simulink model "sm_car_"  (R2026b)
settings: Solver=ode23t  StopTime=100  MaxStep=0.4  AbsTol=1e-3  EnableMultiTasking=on
PreLoadFcn:
  | % Due to usability issue in Repeating Sequence block
  | warning('off','Simulink:Masking:Invalid');
  | 
  | % Eliminate unnecessary warnings in inactive variants
  | % Warnings generated only if you click through inactive variant
  | warning('off','MATLAB:nonExistentField');
  | warning('off','Simulink:Parameters:BlkParamUndefined');
PostLoadFcn:
  | set_param([bdroot '/Vehicle'],'popup_trailer','Off')
  | warning('off','sm:sli:setup:compile:LocalSolverNotSupported')
  | %sm_car_config_maneuver(bdroot,'WOT Braking');
  | sm_car_config_vehicle(bdroot,'false');
  | sm_car_config_logging(bdroot);
InitFcn:
  | sm_car_config_camera;
  | Vehicle = sm_car_vehcfg_checkConfig(Vehicle);
  | sm_car_check_tire_model(bdroot);
StartFcn:
  | tic;
StopFcn:
  | Elapsed_Sim_Time = toc;
  | % disp(['Elapsed Sim Time = ' num2str(Elapsed_Sim_Time)]);
undefined symbols (not defined in the file or in its folder): acc_theta, accel_ramp_rate, Axle1D, AxleIn, Camera, Control, Driver, Init, Maneuver, Pedal, Scene, ShaftL1, ShaftL2, ShaftR1, ShaftR2, Visual, X, xy_data_car_side, Y, Z
libraries: sm_lib x290, fl_lib x171, nesl_utility x144, simulink x60, simulink_extras x14, sdl_lib x14, SimscapeFluids_lib x7, Damper_Element x4, Tire_1x2x x4, ee_lib x3, Scene_Utilities x3, sharedTrackingLibrary x2
(part 6 of 22)

== system sm_car_/Controller/TrqVec_FLC/Power Control ==
  rAccelPedal : Inport
  VehBus : Inport  Port=2
  aSteerWheel : Inport  Port=3
  Bus Creator : BusCreator  Inputs=2
  Bus Selector : BusSelector  OutputSignals=Chassis.Body.CG.vx,Chassis.Body.CG.gy,Chassis.Body.CG.nYaw,Power.MotorL2.w,Power.MotorR2.w
  Gain : Gain  Gain=max(Control.MotorTrq)
  Gain1 : Gain  Gain=max(Control.MotorTrq)
  Gain2 : Gain  Gain=1/9.80665
  TV_FLC : Subsystem  TreatAsAtomicUnit=on  ReferencedSubsystem=TV_FLC  StrWheelRatio=Control.StrWheelRatio  Ku=Control.UndersteerGradient  L=Control.Wheelbase  rwheel=Control.WheelRad  Gr=Control.GearRatio  fis=Control.FuzzySystem  Kp=250  tr=Control.RearTrack  alpha_max=Control.SlipTh  MotorT=Control.MotorTrq  MotorW=Control.MotorW  F=Control.F  Tmax=max(Control.MotorTrq)
  Power : Outport  VectorParamsAs1DForOutWhenUnconnected=off
  wires:
  VehBus/1 -> Bus Selector/1
  Bus Selector/1 -> TV_FLC/2  "<vx>"
  Bus Selector/2 -> Gain2/1  "<gy>"
  Bus Selector/3 -> TV_FLC/4  "<nYaw>"
  Bus Selector/4 -> TV_FLC/5  "<w>"
  Bus Selector/5 -> TV_FLC/6  "<w>"
  rAccelPedal/1 -> TV_FLC/7  "Throttle[~]"
  Bus Creator/1 -> Power/1
  TV_FLC/1 -> Gain/1  "MMotorL2Demand"
  TV_FLC/2 -> Gain1/1  "MMotorR2Demand"
  Gain/1 -> Bus Creator/1  "MMotorL2Demand"
  Gain1/1 -> Bus Creator/2  "MMotorR2Demand"
  Gain2/1 -> TV_FLC/3
  aSteerWheel/1 -> TV_FLC/1

== system sm_car_/Controller/TrqVec_FLC/Spring Damper ==
  Bus Creator : BusCreator  Inputs=4
  Bus Creator1 : BusCreator  Inputs=4
  Constant : Constant  Value=[0 0 0 0]
  Constant1 : Constant  Value=[0 0 0 0]
  Demux : Demux
  Demux1 : Demux
  Damper : Outport  VectorParamsAs1DForOutWhenUnconnected=off
  Spring : Outport  Port=2  VectorParamsAs1DForOutWhenUnconnected=off
  wires:
  Constant/1 -> Demux/1
  Demux/3 -> Bus Creator/3  "L2"
  Demux/4 -> Bus Creator/4  "R2"
  Demux/1 -> Bus Creator/1  "L1"
  Demux/2 -> Bus Creator/2  "R1"
  Demux1/2 -> Bus Creator1/2  "R1"
  Demux1/1 -> Bus Creator1/1  "L1"
  Demux1/4 -> Bus Creator1/4  "R2"
  Demux1/3 -> Bus Creator1/3  "L2"
  Constant1/1 -> Demux1/1
  Bus Creator1/1 -> Damper/1  "Damper"
  Bus Creator/1 -> Spring/1  "Spring"

== system sm_car_/Controller/TrqVec_FLC/Susp ==
  aSteerWheel : Inport
  vx : Inport  Port=2
  1-D Lookup Table : Lookup_n-D  NumberOfTableDimensions=1  BreakpointsForDimension1=Steer.Gain.vVehicle.Value  Table=Steer.Gain.n.Value  InterpMethod=Linear Lagrange  InternalRulePriority=Speed  RndMeth=Simplest
  Bus Creator{1..4} (4 alike) : BusCreator  Inputs=1
  Gain : Gain  Gain=3.6
  Product : Product
  Saturation : Saturate  UpperLimit=Steer.Limits.aUpper.Value  LowerLimit=Steer.Limits.aLower.Value  LinearizeAsGain=off  ZeroCross=off
  Transfer Fcn (with initial states) : simulink_extras/Additional Linear/Transfer Fcn (with initial states)  N=[1]  D="[1/Steer.fActuatorCutoff.Value  1]"  X0=-1
  SuspA1 : Outport  VectorParamsAs1DForOutWhenUnconnected=off
  SuspA2 : Outport  Port=2  VectorParamsAs1DForOutWhenUnconnected=off
  wires:
  Bus Creator4/1 -> Bus Creator1/1  "Steer"
  Bus Creator2/1 -> Bus Creator3/1  "Steer"
  Bus Creator3/1 -> SuspA2/1  "SuspA2"
  Bus Creator1/1 -> SuspA1/1  "SuspA1"
  aSteerWheel/1 -> Product/1, Bus Creator4/1  "aSteerWheel"
  Saturation/1 -> Bus Creator2/1  "aSteerWheel"
  vx/1 -> Gain/1
  Transfer Fcn (with initial states)/1 -> Product/2
  Product/1 -> Saturation/1
  Gain/1 -> 1-D Lookup Table/1
  1-D Lookup Table/1 -> Transfer Fcn (with initial states)/1

== system sm_car_/Controller/TrqVec_FLC_V2/Brake Control ==
  "rBrakePedal " : Inport
  "VehBus " : Inport  Port=2
  Pedal : Subsystem  VariantControl=Pedal
  " Brakes" : Outport  VectorParamsAs1DForOutWhenUnconnected=off

== system sm_car_/Controller/TrqVec_FLC_V2/Driveline Control ==
  Bus Creator : BusCreator  Inputs=1
  Constant : Constant  Value=0
  Driveline : Outport  VectorParamsAs1DForOutWhenUnconnected=off
  wires:
  Constant/1 -> Bus Creator/1  "placeholder"
  Bus Creator/1 -> Driveline/1  "Driveline"

== system sm_car_/Controller/TrqVec_FLC_V2/Power Control ==
  rAccelPedal : Inport
  VehBus : Inport  Port=2
  aSteerWheel : Inport  Port=3
  Bus Creator : BusCreator  Inputs=2
  Bus Selector : BusSelector  OutputSignals=Chassis.Body.CG.vx,Chassis.Body.CG.gx,Chassis.Body.CG.gy,Chassis.Body.CG.nYaw,Chassis.SuspA2.LinkageL.Upright.Upright.w,Chassis.SuspA2.LinkageR.Upright.Upright.w,Chassis.Body.CG.vy
  Controler type : Constant  Value=2
  Gain : Gain  Gain=max(Control.MotorTrq)
  Gain1 : Gain  Gain=max(Control.MotorTrq)
  Gain2 : Gain  Gain=1/9.80665
  TV FLC V2 : Subsystem  TreatAsAtomicUnit=on  ReferencedSubsystem=TV_FLC_V2  MotorT=Control.MotorTrq  Gr=Control.GearRatio  MotorW=Control.MotorW  rwheel=Control.WheelRad  tr=Control.RearTrack  a=Control.FrontTrackToCG  a_cop=Control.FrontTrackToCoP  Af=Control.FrontalArea  cd=Control.LiftCoef  g=Control.GravitationalAcc  ro=Control.AirDensity  m=Control.Mass  h_CG=Control.CGHeight  L=Control.Wheelbase  Gain=Control.StrWheelRatio  Ku=Control.UndersteerGradient  F=Control.F  P=Control.Proportional_P  I=Control.Integral_I  D=Control.Derivative_D  N=Control.Filter_N  Load_Ref=Control.LoadRef  Slip_Ref=Control.SlipRef  FIS_1=Control.FuzzySystem_1  FIS_2=Control.FuzzySystem_2  FIS_3=Control.FuzzySystem_3  vx_th=Control.ActivationVelocity  Tmax=max(Control.MotorTrq)  C_alpha_F=Control.CalphaF
  Power : Outport  VectorParamsAs1DForOutWhenUnconnected=off
  wires:
  aSteerWheel/1 -> TV FLC V2/1
  Gain2/1 -> TV FLC V2/4
  Gain1/1 -> Bus Creator/2  "MMotorR2Demand"
  Gain/1 -> Bus Creator/1  "MMotorL2Demand"
  TV FLC V2/2 -> Gain1/1  "MMotorR2Demand"
  TV FLC V2/1 -> Gain/1  "MMotorL2Demand"
  Bus Creator/1 -> Power/1
  rAccelPedal/1 -> TV FLC V2/9  "Throttle[~]"
  Bus Selector/6 -> TV FLC V2/7  "<w>"
  Bus Selector/5 -> TV FLC V2/6  "<w>"
  Bus Selector/4 -> TV FLC V2/5  "<nYaw>"
  Bus Selector/3 -> Gain2/1  "<gy>"
  Bus Selector/1 -> TV FLC V2/2  "<vx>"
  VehBus/1 -> Bus Selector/1
  Bus Selector/2 -> TV FLC V2/3  "<gx>"
  Bus Selector/7 -> TV FLC V2/8  "<vy>"
  Controler type/1 -> TV FLC V2/10

== system sm_car_/Controller/TrqVec_FLC_V2/Spring Damper ==
  Bus Creator : BusCreator  Inputs=4
  Bus Creator1 : BusCreator  Inputs=4
  Constant : Constant  Value=[0 0 0 0]
  Constant1 : Constant  Value=[0 0 0 0]
  Demux : Demux
  Demux1 : Demux
  Damper : Outport  VectorParamsAs1DForOutWhenUnconnected=off
  Spring : Outport  Port=2  VectorParamsAs1DForOutWhenUnconnected=off
  wires:
  Bus Creator/1 -> Spring/1  "Spring"
  Bus Creator1/1 -> Damper/1  "Damper"
  Constant1/1 -> Demux1/1
  Demux1/3 -> Bus Creator1/3  "L2"
  Demux1/4 -> Bus Creator1/4  "R2"
  Demux1/1 -> Bus Creator1/1  "L1"
  Demux1/2 -> Bus Creator1/2  "R1"
  Demux/2 -> Bus Creator/2  "R1"
  Demux/1 -> Bus Creator/1  "L1"
  Demux/4 -> Bus Creator/4  "R2"
  Demux/3 -> Bus Creator/3  "L2"
  Constant/1 -> Demux/1

== system sm_car_/Controller/TrqVec_FLC_V2/Susp ==
  aSteerWheel : Inport
  vx : Inport  Port=2
  1-D Lookup Table : Lookup_n-D  NumberOfTableDimensions=1  BreakpointsForDimension1=Steer.Gain.vVehicle.Value  Table=Steer.Gain.n.Value  InterpMethod=Linear Lagrange  InternalRulePriority=Speed  RndMeth=Simplest
  Bus Creator{1..4} (4 alike) : BusCreator  Inputs=1
  Gain : Gain  Gain=3.6
  Product : Product
  Saturation : Saturate  UpperLimit=Steer.Limits.aUpper.Value  LowerLimit=Steer.Limits.aLower.Value  LinearizeAsGain=off  ZeroCross=off
  Transfer Fcn (with initial states) : simulink_extras/Additional Linear/Transfer Fcn (with initial states)  N=[1]  D="[1/Steer.fActuatorCutoff.Value  1]"  X0=-1
  SuspA1 : Outport  VectorParamsAs1DForOutWhenUnconnected=off
  SuspA2 : Outport  Port=2  VectorParamsAs1DForOutWhenUnconnected=off
  wires:
  1-D Lookup Table/1 -> Transfer Fcn (with initial states)/1
  Gain/1 -> 1-D Lookup Table/1
  Product/1 -> Saturation/1
  Transfer Fcn (with initial states)/1 -> Product/2
  vx/1 -> Gain/1
  Saturation/1 -> Bus Creator2/1  "aSteerWheel"
  aSteerWheel/1 -> Bus Creator4/1, Product/1  "aSteerWheel"
  Bus Creator1/1 -> SuspA1/1  "SuspA1"
  Bus Creator3/1 -> SuspA2/1  "SuspA2"
  Bus Creator2/1 -> Bus Creator3/1  "Steer"
  Bus Creator4/1 -> Bus Creator1/1  "Steer"

== system sm_car_/Controller/TrqVec_FLC_V3/Brake Control ==
  "rBrakePedal " : Inport
  "VehBus " : Inport  Port=2
  Pedal : Subsystem  VariantControl=Pedal
  " Brakes" : Outport  VectorParamsAs1DForOutWhenUnconnected=off

== system sm_car_/Controller/TrqVec_FLC_V3/Driveline Control ==
  Bus Creator : BusCreator  Inputs=1
  Constant : Constant  Value=0
  Driveline : Outport  VectorParamsAs1DForOutWhenUnconnected=off
  wires:
  Bus Creator/1 -> Driveline/1  "Driveline"
  Constant/1 -> Bus Creator/1  "placeholder"

== system sm_car_/Controller/TrqVec_FLC_V3/Power Control ==
  rAccelPedal : Inport
  VehBus : Inport  Port=2
  aSteerWheel : Inport  Port=3
  Bus Creator : BusCreator  Inputs=2
  Bus Selector : BusSelector  OutputSignals=Chassis.SuspA2.LinkageL.Upright.Upright.w,Chassis.SuspA2.LinkageR.Upright.Upright.w
  Bus Selector1 : BusSelector  OutputSignals=v_x,a_x,a_y,phi_dot,v_y
  Data Type Conversion{,1..8} (9 alike) : DataTypeConversion  OutDataTypeStr=single  SaturateOnIntegerOverflow=off  RndMeth=Floor
  Data Type Conversion10 : DataTypeConversion  OutDataTypeStr=double  SaturateOnIntegerOverflow=off  RndMeth=Floor
  Data Type Conversion11 : DataTypeConversion  OutDataTypeStr=double  SaturateOnIntegerOverflow=off  RndMeth=Floor
  Gain : Gain  Gain=max(Control.MotorTrq)
  Gain1 : Gain  Gain=max(Control.MotorTrq)
  State Estimation : Subsystem
  TV FLC V3 : Subsystem  TreatAsAtomicUnit=on  ReferencedSubsystem=TV_FLC_V3  MotorT=Control.MotorTrq  Gr=Control.GearRatio  MotorW=Control.MotorW  rwheel=Control.WheelRad  tr=Control.RearTrack  a=Control.FrontTrackToCG  a_cop=Control.FrontTrackToCoP  Af=Control.FrontalArea  cd=Control.LiftCoef  Value=Control.GravitationalAcc  ro=Control.AirDensity  m=Control.Mass  h_CG=Control.CGHeight  L=Control.Wheelbase  StrWhlR=Control.StrWheelRatio  Ku=Control.UndersteerGradient  F=Control.F  Slip_Ctrl_Kp=70  Slip_Ctrl_Ki=150  Slip_Ctrl_Kd=1.5  Slip_Ctrl_Kn=Control.Filter_N  Load_Ref=Control.LoadRef  Slip_Ref=Control.SlipRef  FIS=Control.FuzzySystem  vx_th=Control.ActivationVelocity  Tmax=max(Control.MotorTrq)  C_alpha_F=Control.CalphaF  Slip_Steer_th=10  Kp_TV_Yaw=Control.Kp_Yaw  Kp_TV_Beta=Control.Kp_beta
  Power : Outport  VectorParamsAs1DForOutWhenUnconnected=off
  Out Bus Element : Outport  Port=2  PortName=Meas  Element=DYC
  Out Bus Element1 : Outport  Port=2  PortName=Meas  Element=UKF
  wires:
  VehBus/1 -> State Estimation/2(VehBus), Bus Selector/1
  Bus Selector/1 -> Data Type Conversion5/1  "<w>"
  Bus Selector/2 -> Data Type Conversion6/1  "<w>"
  rAccelPedal/1 -> Data Type Conversion8/1  "Throttle[~]"
  Bus Creator/1 -> Power/1
  TV FLC V3/1 -> Data Type Conversion10/1
  Gain/1 -> Bus Creator/1  "MMotorL2Demand"
  Gain1/1 -> Bus Creator/2  "MMotorR2Demand"
  aSteerWheel/1 -> State Estimation/1(aSteerWheel), Data Type Conversion/1
  TV FLC V3/2 -> Data Type Conversion11/1
  Data Type Conversion/1 -> TV FLC V3/1
  Data Type Conversion1/1 -> TV FLC V3/2
  Data Type Conversion2/1 -> TV FLC V3/3
  Data Type Conversion3/1 -> TV FLC V3/4
  Data Type Conversion4/1 -> TV FLC V3/5
  Data Type Conversion5/1 -> TV FLC V3/7
  Data Type Conversion6/1 -> TV FLC V3/8
  Data Type Conversion7/1 -> TV FLC V3/6
  Data Type Conversion8/1 -> TV FLC V3/9
  Data Type Conversion10/1 -> Gain/1
  Data Type Conversion11/1 -> Gain1/1
  TV FLC V3/3 -> Out Bus Element/1
  State Estimation/1(StateEst) -> Bus Selector1/1
  Bus Selector1/1 -> Data Type Conversion1/1  "<v_x>"
  Bus Selector1/4 -> Data Type Conversion4/1  "<phi_dot>"
  Bus Selector1/2 -> Data Type Conversion2/1  "<a_x>"
  Bus Selector1/3 -> Data Type Conversion3/1  "<a_y>"
  Bus Selector1/5 -> Data Type Conversion7/1  "<v_y>"
  State Estimation/2(Meas) -> Out Bus Element1/1  "Estimation"

== system sm_car_/Controller/TrqVec_FLC_V3/Spring Damper ==
  Bus Creator : BusCreator  Inputs=4
  Bus Creator1 : BusCreator  Inputs=4
  Constant : Constant  Value=[0 0 0 0]
  Constant1 : Constant  Value=[0 0 0 0]
  Demux : Demux
  Demux1 : Demux
  Damper : Outport  VectorParamsAs1DForOutWhenUnconnected=off
  Spring : Outport  Port=2  VectorParamsAs1DForOutWhenUnconnected=off
  wires:
  Constant/1 -> Demux/1
  Demux/3 -> Bus Creator/3  "L2"
  Demux/4 -> Bus Creator/4  "R2"
  Demux/1 -> Bus Creator/1  "L1"
  Demux/2 -> Bus Creator/2  "R1"
  Demux1/2 -> Bus Creator1/2  "R1"
  Demux1/1 -> Bus Creator1/1  "L1"
  Demux1/4 -> Bus Creator1/4  "R2"
  Demux1/3 -> Bus Creator1/3  "L2"
  Constant1/1 -> Demux1/1
  Bus Creator1/1 -> Damper/1  "Damper"
  Bus Creator/1 -> Spring/1  "Spring"

== system sm_car_/Controller/TrqVec_FLC_V3/Susp ==
  aSteerWheel : Inport
  vx : Inport  Port=2
  1-D Lookup Table : Lookup_n-D  NumberOfTableDimensions=1  BreakpointsForDimension1=Steer.Gain.vVehicle.Value  Table=Steer.Gain.n.Value  InterpMethod=Linear Lagrange  InternalRulePriority=Speed  RndMeth=Simplest
  Bus Creator{1..4} (4 alike) : BusCreator  Inputs=1
  Gain : Gain  Gain=3.6
  Product : Product
  Saturation : Saturate  UpperLimit=Steer.Limits.aUpper.Value  LowerLimit=Steer.Limits.aLower.Value  LinearizeAsGain=off  ZeroCross=off
  Transfer Fcn (with initial states) : simulink_extras/Additional Linear/Transfer Fcn (with initial states)  N=[1]  D="[1/Steer.fActuatorCutoff.Value  1]"  X0=-1
  SuspA1 : Outport  VectorParamsAs1DForOutWhenUnconnected=off
  SuspA2 : Outport  Port=2  VectorParamsAs1DForOutWhenUnconnected=off
  wires:
  Bus Creator4/1 -> Bus Creator1/1  "Steer"
  Bus Creator2/1 -> Bus Creator3/1  "Steer"
  Bus Creator3/1 -> SuspA2/1  "SuspA2"
  Bus Creator1/1 -> SuspA1/1  "SuspA1"
  aSteerWheel/1 -> Product/1, Bus Creator4/1  "aSteerWheel"
  Saturation/1 -> Bus Creator2/1  "aSteerWheel"
  vx/1 -> Gain/1
  Transfer Fcn (with initial states)/1 -> Product/2
  Product/1 -> Saturation/1
  Gain/1 -> 1-D Lookup Table/1
  1-D Lookup Table/1 -> Transfer Fcn (with initial states)/1

== system sm_car_/Driver/Closed Loop/Driver ==
  vx : Inport
  Ref : Inport  Port=2
  CurPose : Inport  Port=3
  Abs : Abs  SaturateOnIntegerOverflow=off
  Bus Creator5 : BusCreator  Inputs=4
  Bus Selector1 : BusSelector  OutputSignals=vTarget
  Constant : Constant
  Constant1 : Constant  Value=0.8
  Constant9 : Constant  Value=0
  Filter Steer Cmd : TransferFcn  Numerator=[5.7]  Denominator=[1/Driver.Lateral.fSteerCutoff.Value 1]
  Gain4 : Gain  Gain=pi/180
  Get Pose : Subsystem
  Lateral Controller Stanley : drivingvehiclecontroller/Lateral Controller Stanley  ModelType=Kinematic bicycle model  PositionGainF=0.7  PositionGainR=Driver.Lateral.Stanley.NForward.Value  YawRateGain=0.2  DelayGain=0.2  VehicleMass=1575  Lf=1.2  Lr=1.6  TireStiffness=19000  Wheelbase=1.578  MaxSteeringAngle=27
  Longitudinal Driver : autolibshared/Longitudinal Driver  extAccelOvr=off  extDecelOvr=off  extAccelHld=off  extDecelHld=off  extAccelZero=off  extDecelZero=off  cntrlType=Predictive  shftType=None  velUnits=m/s  gearOut=off  Kp=15  Ki=1  Kff=.05  Kg=.01  VehVelVec=[0 100]  KffVec=[.1 .1]  KpVec=[10 10]  KiVec=[5 5]  KgVec=[0 0]  m=320  Kpt=Driver.Long.FTractive.Value  tau=Driver.Long.tDriver.Value  L=3  aR=Driver.Long.NDragRoll.Value  bR=Driver.Long.NDragAero.Value  cR=Driver.Long.NDragAero.Value  g=Driver.Long.gGravity.Value  vnom=100  Kaw=.1  tauerr=.03  tauPt=2  GearInit=0  tShift=.1  pdlVec=[0.1 0.4 0.5 0.9]  upShftTbl=[-1 12.9375 26.4375 39.9375 51.18749999999999 62.4375 72.84375 83.25;-1 16.3125 29.8125 43.3125 54.5624 65.8125 76.78125 87.75;-1 19.6875 33.1875 46.68749999999999 57.9375 69.1875 80.71875 92.25;-1 33 52.5 77.25 100.5 138.75 161.875 185]  dwnShftTbl=[1 9.5625 23.0625 36.5625 47.8125 59.0625 68.90625 78.75;1 12.9375 26.4375 39.9375 51.18749999999999 62.4375 72.84375 83.25;1 16.3125 29.8125 43.3125 54.562499 65.8125 76.78125 87.75;1 19.6875 33.1875 46.68749999999999 57.9375 69.1875 80.71875 92.25]  tClutch=.5  tRev=.5  tPark=120  aMode=1  UpGearVec="[0  1  2  3  4  5  6  7]"  DownGearVec="[1  2  3  4  5  6  7  8]"
  Saturation : Saturate  UpperLimit=inf  LowerLimit=1e-9  ZeroCross=off
  Saturation1 : Saturate  UpperLimit=1  LowerLimit=0  ZeroCross=off
  Saturation2 : Saturate  UpperLimit=1  LowerLimit=0  ZeroCross=off
  Scope : Scope
      settings: ActiveDisplayYMinimum=-1  ActiveDisplayYMaximum=1  DataLoggingVariableName=ScopeData8
  Terminator : Terminator
  Terminator4 : Terminator
  Transfer Fcn : TransferFcn  Denominator=[1/(Driver.Long.fAccelCutoff.Value) 1]
  Transfer Fcn1 : TransferFcn  Denominator=[1/(Driver.Long.fBrakeCutoff.Value) 1]
  DrvBus : Outport  VectorParamsAs1DForOutWhenUnconnected=off
  wires:
  Constant/1 -> Lateral Controller Stanley/4
  Saturation/1 -> Lateral Controller Stanley/3
  Filter Steer Cmd/1 -> Bus Creator5/2  "aSteerWheel"
  Get Pose/1(RefPose) -> Lateral Controller Stanley/1
  Ref/1 -> Bus Selector1/1, Bus Creator5/1, Get Pose/1(Ref)
  vx/1 -> Longitudinal Driver/2, Abs/1
  Transfer Fcn/1 -> Saturation1/1
  Transfer Fcn1/1 -> Saturation2/1
  Abs/1 -> Saturation/1
  Longitudinal Driver/3 -> Transfer Fcn1/1
  CurPose/1 -> Lateral Controller Stanley/2
  Longitudinal Driver/1 -> Terminator/1
  Lateral Controller Stanley/1 -> Gain4/1
  Bus Selector1/1 -> Longitudinal Driver/1  "<vTarget>"
  Bus Creator5/1 -> DrvBus/1  "DrvBus"
  Constant9/1 -> Longitudinal Driver/3
  Longitudinal Driver/2 -> Transfer Fcn/1
  Saturation1/1 -> Bus Creator5/3  "rAccelPedal"
  Saturation2/1 -> Bus Creator5/4  "rBrakePedal"
  Constant1/1 -> Terminator4/1  "rAccelPedal"
  Gain4/1 -> Scope/1, Filter Steer Cmd/1

== system sm_car_/Driver/Closed Loop/Driver Override ==
  In : Inport
  None : Subsystem  VariantControl=None
  Override : Subsystem  VariantControl=Override
  DrvBus : Outport

== system sm_car_/Driver/Closed Loop/Maneuver ==
  VehBus : Inport
  Override : Inport  Port=2
  Bus Creator : BusCreator  Inputs=7
  Bus Selector : BusSelector  OutputSignals=World.x,World.y,World.z,World.aRoll,World.aPitch,World.aYaw,Chassis.Body.CG.vx
  Bus Selector1 : BusSelector  OutputSignals=x,y,z,vx
  Constant : Constant  Value=-1
  Constant6 : Constant  Value=Maneuver.Trajectory.xTrajectory.Value
  Constant8 : Constant  Value=Maneuver.Trajectory.aYaw.Value
  Count Lap : Subsystem
  MATLAB Function : MATLAB Function  SystemSampleTime=0.1
  Max Lateral Distance (m) : Constant  Value=Maneuver.xMaxLat.Value
  Memory : Memory  InitialCondition=-1
  Min Target Speed (m/s) : Constant  Value=Maneuver.vMinTarget.Value
  Mux : Mux  Inputs=3
  Mux1 : Mux  Inputs=3
  PoseTargetVisual : Subsystem
  Switch : Switch  Criteria=u2 > Threshold  SaturateOnIntegerOverflow=off  InputSameDT=off
  Target Speed Gain : Constant  Value=Value
  Window of Points to Check : Constant  Value=10
  preview distance : Lookup_n-D  NumberOfTableDimensions=1  BreakpointsForDimension1=Maneuver.xPreview.v.Value  Table=Maneuver.xPreview.x.Value  InternalRulePriority=Speed  RndMeth=Simplest
  vx override : Subsystem
  window only : Constant
  x override : Subsystem
  y override : Subsystem
  z override : Subsystem
  Ref : Outport  VectorParamsAs1DForOutWhenUnconnected=off
  CurPose : Outport  Port=2  VectorParamsAs1DForOutWhenUnconnected=off
  simres : Outport  Port=3  VectorParamsAs1DForOutWhenUnconnected=off
  wires:
  Bus Selector1/1 -> x override/1(x)  "<x>"
  Bus Selector1/2 -> y override/1(y)  "<y>"
  Bus Selector1/3 -> z override/1(z)  "<z>"
  vx override/1(vx_ovr) -> MATLAB Function/7(speed)
  Bus Selector1/4 -> vx override/1(vx)  "<vx>"
  Override/1 -> Bus Selector1/1
  z override/1(z_ovr) -> MATLAB Function/5(posz)
  MATLAB Function/2(ref_z) -> PoseTargetVisual/4(ref_z)
  Memory/1 -> Switch/1
  window only/1 -> Switch/2
  Constant/1 -> Switch/3
  Switch/1 -> MATLAB Function/14(idx_ptMin_prev)
  MATLAB Function/9(idx_ptMin) -> Memory/1
  Window of Points to Check/1 -> MATLAB Function/6(xywin)
  MATLAB Function/10(simres) -> simres/1
  MATLAB Function/6(vTarget) -> Bus Creator/6  "vTarget"
  Bus Creator/1 -> Ref/1  "Reference"
  MATLAB Function/1(ad) -> Count Lap/1(ad), PoseTargetVisual/1(dist), Bus Creator/2  "dist"
  MATLAB Function/5(ref_ayaw) -> Bus Creator/5, PoseTargetVisual/5(ref_ayaw)  "ayaw"
  MATLAB Function/4(ref_y) -> Bus Creator/4, PoseTargetVisual/3(ref_y)  "y"
  VehBus/1 -> Bus Selector/1
  preview distance/1 -> MATLAB Function/10(pd)
  MATLAB Function/7(cp) -> CurPose/1  "CurPose"
  x override/1(x_ovr) -> MATLAB Function/3(posx)
  MATLAB Function/3(ref_x) -> Bus Creator/3, PoseTargetVisual/2(ref_x)  "x"
  Bus Selector/2 -> Mux/2  "<y>"
  y override/1(y_ovr) -> MATLAB Function/4(posy)
  Bus Selector/3 -> Mux/3  "<z>"
  Mux/1 -> MATLAB Function/1(p)
  Constant6/1 -> MATLAB Function/9(dist)
  Bus Selector/5 -> Mux1/2  "<aPitch>"
  Mux1/1 -> MATLAB Function/2(q)
  Bus Selector/7 -> preview distance/1  "<vx>"
  Constant8/1 -> MATLAB Function/8(yaw)
  Bus Selector/4 -> Mux1/1  "<aRoll>"
  Bus Selector/6 -> Mux1/3  "<aYaw>"
  Bus Selector/1 -> Mux/1  "<x>"
  Max Lateral Distance (m)/1 -> MATLAB Function/11(maxld)
  Target Speed Gain/1 -> MATLAB Function/13(speedGain)
  Min Target Speed (m/s)/1 -> MATLAB Function/12(minSpd)
  MATLAB Function/8(ld) -> Bus Creator/7  "latdev"
  Count Lap/1(lapC) -> Bus Creator/1  "nLap"

== system sm_car_/Driver/Closed Loop/Override ==
  "dist " : Inport
  "Obs " : Inport  Port=2
  None : Subsystem  VariantControl=None  mask(No Driver Override){override=Scene.Mallory_Park_Obstacle.Override}
      mask prompts: override "Override parameters (structure)"
      mask help: Driver commands are not overridden, regardless of inputs to subsystem.
  " Ovr" : Outport  VectorParamsAs1DForOutWhenUnconnected=off

== system sm_car_/Driver/Closed Loop/Scopes ==
  <vx> : Inport
  Ref : Inport  Port=2
  CurPose : Inport  Port=3
  DrvBus : Inport  Port=4
  Bus Selector : BusSelector  OutputSignals=vTarget
  Bus Selector1 : BusSelector  OutputSignals=aSteerWheel,rAccelPedal,rBrakePedal
  Compare vx to Target : Scope  NumInputPorts=2
      settings: ActiveDisplayYMinimum=-4.79181  ActiveDisplayYMaximum=0.54534
  RefPose : Scope
      settings: ActiveDisplayYMinimum=-598.75829  ActiveDisplayYMaximum=469.37365
  Scope1 : Scope  NumInputPorts=3
      settings: ActiveDisplayYMinimum=-1.19495  ActiveDisplayYMaximum=0.13277  DataLoggingVariableName=ScopeData2
  wires:
  DrvBus/1 -> Bus Selector1/1
  Bus Selector1/1 -> Scope1/1  "<aSteerWheel>"
  Bus Selector1/2 -> Scope1/2  "<rAccelPedal>"
  <vx>/1 -> Compare vx to Target/1
  Bus Selector1/3 -> Scope1/3  "<rBrakePedal>"
  CurPose/1 -> RefPose/1
  Bus Selector/1 -> Compare vx to Target/2  "<vTarget>"
  Ref/1 -> Bus Selector/1

== system sm_car_/Driver/Closed Loop1/Driver ==
  vx : Inport
  Ref : Inport  Port=2
  CurPose : Inport  Port=3
  Abs : Abs  SaturateOnIntegerOverflow=off
  Bus Creator5 : BusCreator  Inputs=4
  Bus Selector1 : BusSelector  OutputSignals=vTarget
  Constant : Constant
  Constant1 : Constant  Value=0.8
  Constant9 : Constant  Value=0
  Filter Steer Cmd : TransferFcn  Numerator=[6.5]  Denominator=[1/Driver.Lateral.fSteerCutoff.Value 1]
  Gain4 : Gain  Gain=pi/180
  Get Pose : Subsystem
  Lateral Controller Stanley : drivingvehiclecontroller/Lateral Controller Stanley  ModelType=Kinematic bicycle model  PositionGainF=0.7  PositionGainR=Driver.Lateral.Stanley.NForward.Value  YawRateGain=0.2  DelayGain=0.2  VehicleMass=1575  Lf=1.2  Lr=1.6  TireStiffness=19000  Wheelbase=1.578  MaxSteeringAngle=27
  Longitudinal Driver : autolibshared/Longitudinal Driver  extAccelOvr=off  extDecelOvr=off  extAccelHld=off  extDecelHld=off  extAccelZero=off  extDecelZero=off  cntrlType=Predictive  shftType=None  velUnits=m/s  gearOut=off  Kp=15  Ki=1  Kff=.05  Kg=.01  VehVelVec=[0 100]  KffVec=[.1 .1]  KpVec=[10 10]  KiVec=[5 5]  KgVec=[0 0]  m=320  Kpt=Driver.Long.FTractive.Value  tau=Driver.Long.tDriver.Value  L=3  aR=Driver.Long.NDragRoll.Value  bR=Driver.Long.NDragAero.Value  cR=Driver.Long.NDragAero.Value  g=Driver.Long.gGravity.Value  vnom=100  Kaw=.1  tauerr=.03  tauPt=2  GearInit=0  tShift=.1  pdlVec=[0.1 0.4 0.5 0.9]  upShftTbl=[-1 12.9375 26.4375 39.9375 51.18749999999999 62.4375 72.84375 83.25;-1 16.3125 29.8125 43.3125 54.5624 65.8125 76.78125 87.75;-1 19.6875 33.1875 46.68749999999999 57.9375 69.1875 80.71875 92.25;-1 33 52.5 77.25 100.5 138.75 161.875 185]  dwnShftTbl=[1 9.5625 23.0625 36.5625 47.8125 59.0625 68.90625 78.75;1 12.9375 26.4375 39.9375 51.18749999999999 62.4375 72.84375 83.25;1 16.3125 29.8125 43.3125 54.562499 65.8125 76.78125 87.75;1 19.6875 33.1875 46.68749999999999 57.9375 69.1875 80.71875 92.25]  tClutch=.5  tRev=.5  tPark=120  aMode=1  UpGearVec="[0  1  2  3  4  5  6  7]"  DownGearVec="[1  2  3  4  5  6  7  8]"
  Predictive Driver : vehdynlibdriver/Predictive Driver  extAccelOvr=off  extDecelOvr=off  extAccelHld=off  extDecelHld=off  extAccelZero=off  extDecelZero=off  extSteerOvr=off  extSteerHld=off  extSteerZero=off  cntrlType=Predictive  cntrlTypeLat=Stanley  shftType=None  coordMode=SAE J670 (Z-down)  refType=Reference pose  velUnits=m/s  angUnits=rad  gearOut=off  steerOut=on  Kp=10  Ki=5  Kff=.1  Kg=0  VehVelVec=[0 100]  KffVec=[.1 .1]  KpVec=[10 10]  KiVec=[5 5]  KgVec=[0 0]  vnom=5  Kaw=1  tauerr=.01  tau=0.1  L=0.3  Kpt=3000  aR=200  bR=2.5  cR=.5  g=9.81  vecPose=on  dynamMode=off  PositionGainF=1  PositionGainR=2.5  YawRateGain=.2  DelayGain=.2  enableDrift=off  BetaRef=20*pi/180  KpBeta=1  KpDrift=2  KdDrift=1  KpPsi=6  KOmega=30  tOmega=1  a=0.8232  b=0.7518  m=319  Cy_f=46000  Cy_r=70933  I=4013  Ksteer=6.56  theta=34*pi/180  Idl=3  Re=.3  lambda_mu=1  GearInit=0  tShift=.1  pdlVec=[0.1 0.4 0.5 0.9]  upShftTbl=[-1 12.9375 26.4375 39.9375 51.18749999999999 62.4375 72.84375 83.25;-1 16.3125 29.8125 43.3125 54.5624 65.8125 76.78125 87.75;-1 19.6875 33.1875 46.68749999999999 57.9375 69.1875 80.71875 92.25;-1 33 52.5 77.25 100.5 138.75 161.875 185]  dwnShftTbl=[-1 12.9375 26.4375 39.9375 51.18749999999999 62.4375 72.84375 83.25;-1 16.3125 29.8125 43.3125 54.5624 65.8125 76.78125 87.75;-1 19.6875 33.1875 46.68749999999999 57.9375 69.1875 80.71875 92.25;-1 33 52.5 77.25 100.5 138.75 161.875 185]  tClutch=.5  tRev=.5  tPark=120  UpGearVec="[0  1  2  3  4  5  6  7]"  DownGearVec="[1  2  3  4  5  6  7  8]"  aMode=2
  Saturation : Saturate  UpperLimit=inf  LowerLimit=1e-9  ZeroCross=off
  Saturation1 : Saturate  UpperLimit=1  LowerLimit=0  ZeroCross=off
  Saturation2 : Saturate  UpperLimit=1  LowerLimit=0  ZeroCross=off
  Scope : Scope
      settings: ActiveDisplayYMinimum=-1  ActiveDisplayYMaximum=1  DataLoggingVariableName=ScopeData8
  Terminator : Terminator
  Terminator1 : Terminator
  Terminator4 : Terminator
  Transfer Fcn : TransferFcn  Denominator=[1/(Driver.Long.fAccelCutoff.Value) 1]
  Transfer Fcn1 : TransferFcn  Denominator=[1/(Driver.Long.fBrakeCutoff.Value) 1]
  Transfer Fcn2 : TransferFcn  Denominator=[1/(Driver.Long.fAccelCutoff.Value) 1]
  Transfer Fcn3 : TransferFcn  Denominator=[1/(Driver.Long.fBrakeCutoff.Value) 1]
  Trasform Pose : Subsystem
  DrvBus : Outport  VectorParamsAs1DForOutWhenUnconnected=off
  wires:
  Gain4/1 -> Filter Steer Cmd/1, Scope/1
  Constant1/1 -> Terminator4/1  "rAccelPedal"
  Saturation2/1 -> ?  "rBrakePedal"
  Saturation1/1 -> ?  "rAccelPedal"
  Longitudinal Driver/2 -> Transfer Fcn/1
  Constant9/1 -> Predictive Driver/3
  Bus Creator5/1 -> DrvBus/1  "DrvBus"
  Lateral Controller Stanley/1 -> Gain4/1
  Longitudinal Driver/1 -> Terminator/1
  Longitudinal Driver/3 -> Transfer Fcn1/1
  Abs/1 -> Saturation/1
  Transfer Fcn1/1 -> Saturation2/1
  Transfer Fcn/1 -> Saturation1/1
  vx/1 -> Predictive Driver/4, Abs/1
  Ref/1 -> Bus Selector1/1, Get Pose/1(Ref), Bus Creator5/1
  Get Pose/1(RefPose) -> Predictive Driver/2
  Filter Steer Cmd/1 -> ?  "aSteerWheel"
  Constant/1 -> Lateral Controller Stanley/4
  Bus Selector1/1 -> Predictive Driver/1  "<vTarget>"
  Predictive Driver/2 -> Bus Creator5/2  "aSteerWheel"
  Predictive Driver/3 -> Transfer Fcn2/1  "rAccelPedal"
  Predictive Driver/4 -> Transfer Fcn3/1  "rBrakePedal"
  Predictive Driver/1 -> Terminator1/1
  Transfer Fcn2/1 -> Bus Creator5/3  "rAccelPedal"
  Transfer Fcn3/1 -> Bus Creator5/4  "rBrakePedal"
  CurPose/1 -> Trasform Pose/1(CurPose)
  Trasform Pose/1(CurrPoseCG) -> Predictive Driver/5

== system sm_car_/Driver/Closed Loop1/Driver Override ==
  In : Inport
  None : Subsystem  VariantControl=None
  Override : Subsystem  VariantControl=Override
  DrvBus : Outport

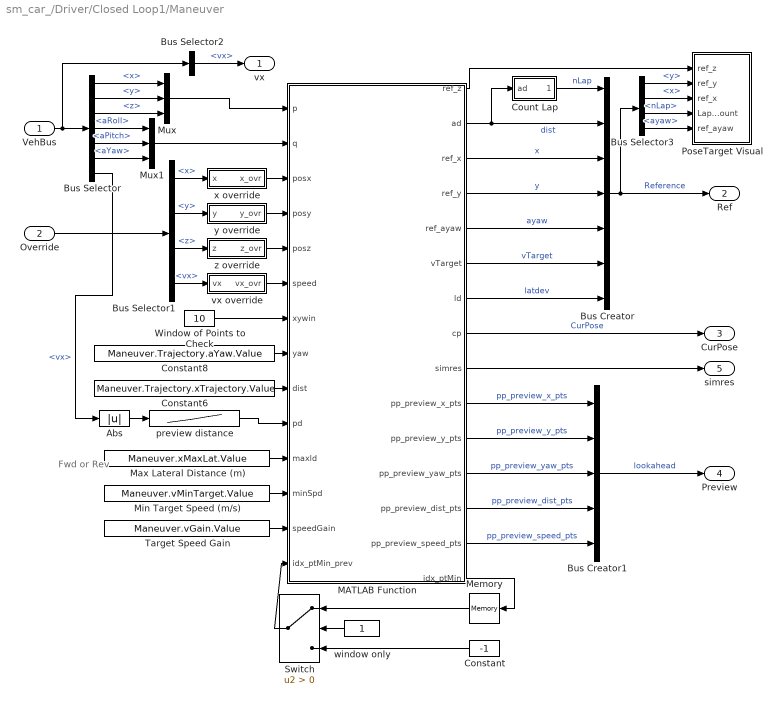
== system sm_car_/Driver/Closed Loop1/Maneuver ==
  note: Fwd or
      | Rev
  VehBus : Inport
  Override : Inport  Port=2
  Abs : Abs  ZeroCross=off  SaturateOnIntegerOverflow=off
  Bus Creator : BusCreator  Inputs=7
  Bus Creator1 : BusCreator  Inputs=5
  Bus Selector : BusSelector  OutputSignals=World.x,World.y,World.z,World.aRoll,World.aPitch,World.aYaw,Chassis.Body.CG.vx
  Bus Selector1 : BusSelector  OutputSignals=x,y,z,vx
  Bus Selector2 : BusSelector  OutputSignals=Chassis.Body.CG.vx
  Bus Selector3 : BusSelector  OutputSignals=y,x,nLap,ayaw
  Constant : Constant  Value=-1
  Constant6 : Constant  Value=Maneuver.Trajectory.xTrajectory.Value
  Constant8 : Constant  Value=Maneuver.Trajectory.aYaw.Value
  Count Lap : Subsystem
  MATLAB Function : MATLAB Function  SystemSampleTime=0.1  mask{nPreviewPoints=Maneuver.nPreviewPoints.Value}
      mask prompts: nPreviewPoints "Number of Preview Points"
  Max Lateral Distance (m) : Constant  Value=Maneuver.xMaxLat.Value
  Memory : Memory  InitialCondition=-1
  Min Target Speed (m/s) : Constant  Value=Maneuver.vMinTarget.Value
  Mux : Mux  Inputs=3
  Mux1 : Mux  Inputs=3
  PoseTarget Visual : Subsystem
  Switch : Switch  Criteria=u2 > Threshold  SaturateOnIntegerOverflow=off  InputSameDT=off
  Target Speed Gain : Constant  Value=Maneuver.vGain.Value
  Window of Points to Check : Constant  Value=10
  preview distance : Lookup_n-D  NumberOfTableDimensions=1  BreakpointsForDimension1=Maneuver.xPreview.v.Value  Table=Maneuver.xPreview.x.Value  InternalRulePriority=Speed  RndMeth=Simplest
  vx override : Subsystem
  window only : Constant
  x override : Subsystem
  y override : Subsystem
  z override : Subsystem
  vx : Outport  VectorParamsAs1DForOutWhenUnconnected=off
  Ref : Outport  Port=2  VectorParamsAs1DForOutWhenUnconnected=off
  CurPose : Outport  Port=3  VectorParamsAs1DForOutWhenUnconnected=off
  Preview : Outport  Port=4  VectorParamsAs1DForOutWhenUnconnected=off
  simres : Outport  Port=5  VectorParamsAs1DForOutWhenUnconnected=off
  wires:
  MATLAB Function/14(pp_preview_speed_pts) -> Bus Creator1/5  "pp_preview_speed_pts"
  MATLAB Function/1(ref_z) -> PoseTarget Visual/1(ref_z)
  Bus Selector3/4 -> PoseTarget Visual/5(ref_ayaw)  "<ayaw>"
  Bus Selector3/3 -> PoseTarget Visual/4(Lap Count)  "<nLap>"
  Bus Selector3/2 -> PoseTarget Visual/3(ref_x)  "<x>"
  Bus Selector3/1 -> PoseTarget Visual/2(ref_y)  "<y>"
  Count Lap/1(lapC) -> Bus Creator/1  "nLap"
  Bus Selector2/1 -> vx/1  "<vx>"
  VehBus/1 -> Bus Selector/1, Bus Selector2/1
  Bus Creator1/1 -> Preview/1  "lookahead"
  MATLAB Function/13(pp_preview_dist_pts) -> Bus Creator1/4  "pp_preview_dist_pts"
  MATLAB Function/12(pp_preview_yaw_pts) -> Bus Creator1/3  "pp_preview_yaw_pts"
  MATLAB Function/11(pp_preview_y_pts) -> Bus Creator1/2  "pp_preview_y_pts"
  MATLAB Function/10(pp_preview_x_pts) -> Bus Creator1/1  "pp_preview_x_pts"
  MATLAB Function/7(ld) -> Bus Creator/7  "latdev"
  Min Target Speed (m/s)/1 -> MATLAB Function/12(minSpd)
  Target Speed Gain/1 -> MATLAB Function/13(speedGain)
  Max Lateral Distance (m)/1 -> MATLAB Function/11(maxld)
  Bus Selector/1 -> Mux/1  "<x>"
  Bus Selector/6 -> Mux1/3  "<aYaw>"
  Bus Selector/4 -> Mux1/1  "<aRoll>"
  Constant8/1 -> MATLAB Function/8(yaw)
  Bus Selector/7 -> Abs/1  "<vx>"
  Mux1/1 -> MATLAB Function/2(q)
  Bus Selector/5 -> Mux1/2  "<aPitch>"
  Constant6/1 -> MATLAB Function/9(dist)
  Mux/1 -> MATLAB Function/1(p)
  Bus Selector/3 -> Mux/3  "<z>"
  y override/1(y_ovr) -> MATLAB Function/4(posy)
  Bus Selector/2 -> Mux/2  "<y>"
  MATLAB Function/3(ref_x) -> Bus Creator/3  "x"
  x override/1(x_ovr) -> MATLAB Function/3(posx)
  MATLAB Function/8(cp) -> CurPose/1  "CurPose"
  preview distance/1 -> MATLAB Function/10(pd)
  MATLAB Function/4(ref_y) -> Bus Creator/4  "y"
  MATLAB Function/5(ref_ayaw) -> Bus Creator/5  "ayaw"
  MATLAB Function/2(ad) -> Count Lap/1(ad), Bus Creator/2  "dist"
  Bus Creator/1 -> Bus Selector3/1, Ref/1  "Reference"
  MATLAB Function/6(vTarget) -> Bus Creator/6  "vTarget"
  MATLAB Function/9(simres) -> simres/1
  Window of Points to Check/1 -> MATLAB Function/7(xywin)
  MATLAB Function/15(idx_ptMin) -> Memory/1
  Switch/1 -> MATLAB Function/14(idx_ptMin_prev)
  Constant/1 -> Switch/3
  window only/1 -> Switch/2
  Memory/1 -> Switch/1
  z override/1(z_ovr) -> MATLAB Function/5(posz)
  Override/1 -> Bus Selector1/1
  Bus Selector1/4 -> vx override/1(vx)  "<vx>"
  vx override/1(vx_ovr) -> MATLAB Function/6(speed)
  Bus Selector1/3 -> z override/1(z)  "<z>"
  Bus Selector1/2 -> y override/1(y)  "<y>"
  Bus Selector1/1 -> x override/1(x)  "<x>"
  Abs/1 -> preview distance/1

== system sm_car_/Driver/Closed Loop1/Override ==
  "dist " : Inport
  "Obs " : Inport  Port=2
  None : Subsystem  VariantControl=None  mask(No Driver Override){override=Scene.Mallory_Park_Obstacle.Override}
      mask prompts: override "Override parameters (structure)"
      mask help: Driver commands are not overridden, regardless of inputs to subsystem.
  " Ovr" : Outport  VectorParamsAs1DForOutWhenUnconnected=off

== system sm_car_/Driver/Closed Loop1/Scopes ==
  <vx> : Inport
  Ref : Inport  Port=2
  CurPose : Inport  Port=3
  DrvBus : Inport  Port=4
  Bus Selector : BusSelector  OutputSignals=vTarget
  Bus Selector1 : BusSelector  OutputSignals=aSteerWheel,rAccelPedal,rBrakePedal
  Compare vx to Target : Scope  NumInputPorts=2
      settings: ActiveDisplayYMinimum=-4.79181  ActiveDisplayYMaximum=0.54534
  RefPose : Scope
      settings: ActiveDisplayYMinimum=-598.75829  ActiveDisplayYMaximum=469.37365
  Scope1 : Scope  NumInputPorts=3
      settings: ActiveDisplayYMinimum=-1.19495  ActiveDisplayYMaximum=0.13277  DataLoggingVariableName=ScopeData2
  wires:
  Ref/1 -> Bus Selector/1
  Bus Selector/1 -> Compare vx to Target/2  "<vTarget>"
  CurPose/1 -> RefPose/1
  Bus Selector1/3 -> Scope1/3  "<rBrakePedal>"
  <vx>/1 -> Compare vx to Target/1
  Bus Selector1/2 -> Scope1/2  "<rAccelPedal>"
  Bus Selector1/1 -> Scope1/1  "<aSteerWheel>"
  DrvBus/1 -> Bus Selector1/1

== system sm_car_/Driver/Open Loop/Open Loop ==
  Bus Creator : BusCreator  Inputs=7
  Bus Creator5 : BusCreator  Inputs=4
  Constant : Constant  Value=10000
  Constant{1..6} (6 alike) : Constant  Value=0
  Input Sequence Accel Pedal : simulink/Sources/Repeating Sequence  rep_seq_t=Maneuver.Accel.t.Value  rep_seq_y=Maneuver.Accel.rPedal.Value
  Input Sequence Brake Pedal : simulink/Sources/Repeating Sequence  rep_seq_t=Maneuver.Brake.t.Value  rep_seq_y=Maneuver.Brake.rPedal.Value
  "Input Sequence Steering Wheel " : simulink/Sources/Repeating Sequence  rep_seq_t=Maneuver.Steer.t.Value  rep_seq_y=Maneuver.Steer.aWheel.Value
  DrvBus : Outport  VectorParamsAs1DForOutWhenUnconnected=off
  wires:
  Constant6/1 -> Bus Creator/7  "nLap"
  Constant/1 -> Bus Creator/1  "dist"
  Bus Creator/1 -> Bus Creator5/1  "Reference"
  Constant4/1 -> Bus Creator/5  "vTarget"
  Constant3/1 -> Bus Creator/4  "ayaw"
  Constant2/1 -> Bus Creator/3  "y"
  Constant5/1 -> Bus Creator/6  "latdev"
  Constant1/1 -> Bus Creator/2  "x"
  Input Sequence Accel Pedal/1 -> Bus Creator5/3  "rAccelPedal"
  "Input Sequence Steering Wheel "/1 -> Bus Creator5/2  "aSteerWheel"
  Input Sequence Brake Pedal/1 -> Bus Creator5/4  "rBrakePedal"
  Bus Creator5/1 -> DrvBus/1  "DrvBus"

== system sm_car_/Road/Mu Scaling by Position/Scaling factors FL ==
  muX : Inport
  muY : Inport  Port=2
  s_LKX : Constant  Value=LKX
  s_LKY : Constant  Value=LKY
  s_LKYC : Constant  Value=LKYC
  s_LKZC : Constant  Value=LKZC
  s_LTR : Constant  Value=LTR
  scaling_vector : Mux  Inputs=7
  scaling : Outport  VectorParamsAs1DForOutWhenUnconnected=off
  wires:
  muX/1 -> scaling_vector/1
  s_LKX/1 -> scaling_vector/2
  muY/1 -> scaling_vector/3
  s_LKY/1 -> scaling_vector/4
  s_LKYC/1 -> scaling_vector/5
  s_LTR/1 -> scaling_vector/6
  s_LKZC/1 -> scaling_vector/7
  scaling_vector/1 -> scaling/1

== system sm_car_/Road/Mu Scaling by Position/Scaling factors FR ==
  muX : Inport
  muY : Inport  Port=2
  s_LKX : Constant  Value=LKX
  s_LKY : Constant  Value=LKY
  s_LKYC : Constant  Value=LKYC
  s_LKZC : Constant  Value=LKZC
  s_LTR : Constant  Value=LTR
  scaling_vector : Mux  Inputs=7
  scaling : Outport  VectorParamsAs1DForOutWhenUnconnected=off
  wires:
  muX/1 -> scaling_vector/1
  s_LKX/1 -> scaling_vector/2
  muY/1 -> scaling_vector/3
  s_LKY/1 -> scaling_vector/4
  s_LKYC/1 -> scaling_vector/5
  s_LTR/1 -> scaling_vector/6
  s_LKZC/1 -> scaling_vector/7
  scaling_vector/1 -> scaling/1

== system sm_car_/Road/Mu Scaling by Position/Scaling factors RL ==
  muX : Inport
  muY : Inport  Port=2
  s_LKX : Constant  Value=LKX
  s_LKY : Constant  Value=LKY
  s_LKYC : Constant  Value=LKYC
  s_LKZC : Constant  Value=LKZC
  s_LTR : Constant  Value=LTR
  scaling_vector : Mux  Inputs=7
  scaling : Outport  VectorParamsAs1DForOutWhenUnconnected=off
  wires:
  muX/1 -> scaling_vector/1
  s_LKX/1 -> scaling_vector/2
  muY/1 -> scaling_vector/3
  s_LKY/1 -> scaling_vector/4
  s_LKYC/1 -> scaling_vector/5
  s_LTR/1 -> scaling_vector/6
  s_LKZC/1 -> scaling_vector/7
  scaling_vector/1 -> scaling/1

== system sm_car_/Road/Mu Scaling by Position/Scaling factors RR ==
  muX : Inport
  muY : Inport  Port=2
  s_LKX : Constant  Value=LKX
  s_LKY : Constant  Value=LKY
  s_LKYC : Constant  Value=LKYC
  s_LKZC : Constant  Value=LKZC
  s_LTR : Constant  Value=LTR
  scaling_vector : Mux  Inputs=7
  scaling : Outport  VectorParamsAs1DForOutWhenUnconnected=off
  wires:
  muX/1 -> scaling_vector/1
  s_LKX/1 -> scaling_vector/2
  muY/1 -> scaling_vector/3
  s_LKY/1 -> scaling_vector/4
  s_LKYC/1 -> scaling_vector/5
  s_LTR/1 -> scaling_vector/6
  s_LKZC/1 -> scaling_vector/7
  scaling_vector/1 -> scaling/1

== system sm_car_/Road/Road Surface Height/None ==
  Chassis : Inport
  Bus Creator : BusCreator  Inputs=4
  Bus Creator1 : BusCreator  Inputs=4
  Constant : Constant  Value=[0 0 0 0]
  Constant{1..4} (4 alike) : Constant  Value=[0 0 1]
  Demux2 : Demux
  Signal Specification1 : SignalSpecification  Unit=m
  Terminator : Terminator
  gz : Outport  VectorParamsAs1DForOutWhenUnconnected=off
  uvec : Outport  Port=2  VectorParamsAs1DForOutWhenUnconnected=off
  wires:
  Bus Creator/1 -> uvec/1  "uvec"
  Constant4/1 -> Bus Creator/4  "R2"
  Constant1/1 -> Bus Creator/1  "L1"
  Constant2/1 -> Bus Creator/2  "R1"
  Constant3/1 -> Bus Creator/3  "L2"
  Demux2/3 -> Bus Creator1/3  "L2"
  Demux2/4 -> Bus Creator1/4  "R2"
  Demux2/2 -> Bus Creator1/2  "R1"
  Bus Creator1/1 -> gz/1  "gz"
  Signal Specification1/1 -> Demux2/1
  Demux2/1 -> Bus Creator1/1  "L1"
  Constant/1 -> Signal Specification1/1
  Chassis/1 -> Terminator/1

== system sm_car_/Scopes/Combined Tire Usage/FL_Fcomb ==
  <Fx> : Inport
  <Fy> : Inport  Port=2
  <Fz> : Inport  Port=3
  <rMuX> : Inport  Port=4
  <rMuY> : Inport  Port=5
  Abs : Abs  SaturateOnIntegerOverflow=off
  Add : Sum
  Add1 : Sum
  Divide : Product  Inputs=*/
  Gain : Gain  Gain=100
  Product : Product
  Product1 : Product
  Safe Division : Bias  Bias=0.01  SaturateOnIntegerOverflow=off
  Square{,1,3..4} (4 alike) : Math  Operator=square
  Square Root : Sqrt
  Square Root1 : Sqrt
  Fcomb% : Outport
  wires:
  Abs/1 -> Fcomb%/1
  Add/1 -> Square Root/1
  Square1/1 -> Add/2
  <Fx>/1 -> Square/1
  <Fz>/1 -> Safe Division/1
  <Fy>/1 -> Square1/1
  Gain/1 -> Abs/1
  Square/1 -> Add/1
  Square Root/1 -> Divide/1
  <rMuX>/1 -> Product/1
  Product1/1 -> Square4/1
  Product/1 -> Square3/1
  Square3/1 -> Add1/1
  Divide/1 -> Gain/1
  Square4/1 -> Add1/2
  Add1/1 -> Square Root1/1
  Square Root1/1 -> Divide/2
  <rMuY>/1 -> Product1/2
  Safe Division/1 -> Product1/1, Product/2

== system sm_car_/Scopes/Combined Tire Usage/FR_Fcomb ==
  <Fx> : Inport
  <Fy> : Inport  Port=2
  <Fz> : Inport  Port=3
  <rMuX> : Inport  Port=4
  <rMuY> : Inport  Port=5
  Abs : Abs  SaturateOnIntegerOverflow=off
  Add : Sum
  Add1 : Sum
  Divide : Product  Inputs=*/
  Gain : Gain  Gain=100
  Product : Product
  Product1 : Product
  Safe Division : Bias  Bias=0.01  SaturateOnIntegerOverflow=off
  Square{,1,3..4} (4 alike) : Math  Operator=square
  Square Root : Sqrt
  Square Root1 : Sqrt
  Fcomb% : Outport
  wires:
  Safe Division/1 -> Product/2, Product1/1
  <rMuY>/1 -> Product1/2
  Square Root1/1 -> Divide/2
  Add1/1 -> Square Root1/1
  Square4/1 -> Add1/2
  Divide/1 -> Gain/1
  Square3/1 -> Add1/1
  Product/1 -> Square3/1
  Product1/1 -> Square4/1
  <rMuX>/1 -> Product/1
  Square Root/1 -> Divide/1
  Square/1 -> Add/1
  Gain/1 -> Abs/1
  <Fy>/1 -> Square1/1
  <Fz>/1 -> Safe Division/1
  <Fx>/1 -> Square/1
  Square1/1 -> Add/2
  Add/1 -> Square Root/1
  Abs/1 -> Fcomb%/1

== system sm_car_/Scopes/Combined Tire Usage/RL_Fcomb ==
  <Fx> : Inport
  <Fy> : Inport  Port=2
  <Fz> : Inport  Port=3
  <rMuX> : Inport  Port=4
  <rMuY> : Inport  Port=5
  Abs : Abs  SaturateOnIntegerOverflow=off
  Add : Sum
  Add1 : Sum
  Divide : Product  Inputs=*/
  Gain : Gain  Gain=100
  Product : Product
  Product1 : Product
  Safe Division : Bias  Bias=0.01  SaturateOnIntegerOverflow=off
  Square{,1,3..4} (4 alike) : Math  Operator=square
  Square Root : Sqrt
  Square Root1 : Sqrt
  Fcomb% : Outport
  wires:
  Abs/1 -> Fcomb%/1
  Add/1 -> Square Root/1
  Square1/1 -> Add/2
  <Fx>/1 -> Square/1
  <Fz>/1 -> Safe Division/1
  <Fy>/1 -> Square1/1
  Gain/1 -> Abs/1
  Square/1 -> Add/1
  Square Root/1 -> Divide/1
  <rMuX>/1 -> Product/1
  Product1/1 -> Square4/1
  Product/1 -> Square3/1
  Square3/1 -> Add1/1
  Divide/1 -> Gain/1
  Square4/1 -> Add1/2
  Add1/1 -> Square Root1/1
  Square Root1/1 -> Divide/2
  <rMuY>/1 -> Product1/2
  Safe Division/1 -> Product1/1, Product/2

== system sm_car_/Scopes/Combined Tire Usage/RR_Fcomb ==
  <Fx> : Inport
  <Fy> : Inport  Port=2
  <Fz> : Inport  Port=3
  <rMuX> : Inport  Port=4
  <rMuY> : Inport  Port=5
  Abs : Abs  SaturateOnIntegerOverflow=off
  Add : Sum
  Add1 : Sum
  Divide : Product  Inputs=*/
  Gain : Gain  Gain=100
  Product : Product
  Product1 : Product
  Safe Division : Bias  Bias=0.01  SaturateOnIntegerOverflow=off
  Square{,1,3..4} (4 alike) : Math  Operator=square
  Square Root : Sqrt
  Square Root1 : Sqrt
  Fcomb% : Outport
  wires:
  Safe Division/1 -> Product/2, Product1/1
  <rMuY>/1 -> Product1/2
  Square Root1/1 -> Divide/2
  Add1/1 -> Square Root1/1
  Square4/1 -> Add1/2
  Divide/1 -> Gain/1
  Square3/1 -> Add1/1
  Product/1 -> Square3/1
  Product1/1 -> Square4/1
  <rMuX>/1 -> Product/1
  Square Root/1 -> Divide/1
  Square/1 -> Add/1
  Gain/1 -> Abs/1
  <Fy>/1 -> Square1/1
  <Fz>/1 -> Safe Division/1
  <Fx>/1 -> Square/1
  Square1/1 -> Add/2
  Add/1 -> Square Root/1
  Abs/1 -> Fcomb%/1

== system sm_car_/Scopes/Lateral Tire Usage/FL_Y ==
  <Fy> : Inport
  <rMuY> : Inport  Port=2
  <Fz> : Inport  Port=3
  Abs : Abs  SaturateOnIntegerOverflow=off
  Divide : Product  Inputs=*/
  Gain : Gain  Gain=100
  Product : Product
  Safe Division : Bias  Bias=0.01  SaturateOnIntegerOverflow=off
  Fy% : Outport
  wires:
  Abs/1 -> Fy%/1
  Divide/1 -> Gain/1
  Product/1 -> Divide/2
  <Fy>/1 -> Divide/1
  <Fz>/1 -> Safe Division/1
  <rMuY>/1 -> Product/1
  Gain/1 -> Abs/1
  Safe Division/1 -> Product/2

== system sm_car_/Scopes/Lateral Tire Usage/FR_Y ==
  <Fy> : Inport
  <rMuY> : Inport  Port=2
  <Fz> : Inport  Port=3
  Abs : Abs  SaturateOnIntegerOverflow=off
  Divide : Product  Inputs=*/
  Gain : Gain  Gain=100
  Product : Product
  Safe Division : Bias  Bias=0.01  SaturateOnIntegerOverflow=off
  Fy% : Outport
  wires:
  Abs/1 -> Fy%/1
  Divide/1 -> Gain/1
  Product/1 -> Divide/2
  <Fy>/1 -> Divide/1
  <Fz>/1 -> Safe Division/1
  <rMuY>/1 -> Product/1
  Gain/1 -> Abs/1
  Safe Division/1 -> Product/2

== system sm_car_/Scopes/Lateral Tire Usage/RL_Y ==
  <Fy> : Inport
  <rMuY> : Inport  Port=2
  <Fz> : Inport  Port=3
  Abs : Abs  SaturateOnIntegerOverflow=off
  Divide : Product  Inputs=*/
  Gain : Gain  Gain=100
  Product : Product
  Safe Division : Bias  Bias=0.01  SaturateOnIntegerOverflow=off
  Fy% : Outport
  wires:
  Safe Division/1 -> Product/2
  Gain/1 -> Abs/1
  <rMuY>/1 -> Product/1
  <Fz>/1 -> Safe Division/1
  <Fy>/1 -> Divide/1
  Product/1 -> Divide/2
  Divide/1 -> Gain/1
  Abs/1 -> Fy%/1

== system sm_car_/Scopes/Lateral Tire Usage/RR_Y ==
  <Fy> : Inport
  <rMuY> : Inport  Port=2
  <Fz> : Inport  Port=3
  Abs : Abs  SaturateOnIntegerOverflow=off
  Divide : Product  Inputs=*/
  Gain : Gain  Gain=100
  Product : Product
  Safe Division : Bias  Bias=0.01  SaturateOnIntegerOverflow=off
  Fy% : Outport
  wires:
  Abs/1 -> Fy%/1
  Divide/1 -> Gain/1
  Product/1 -> Divide/2
  <Fy>/1 -> Divide/1
  <Fz>/1 -> Safe Division/1
  <rMuY>/1 -> Product/1
  Gain/1 -> Abs/1
  Safe Division/1 -> Product/2

== system sm_car_/Scopes/Longitudinal Tire Usage/RL_X ==
  <Fx> : Inport
  <rMuX> : Inport  Port=2
  <Fz> : Inport  Port=3
  Abs : Abs  SaturateOnIntegerOverflow=off
  Add Constant : Bias  Bias=0.01  SaturateOnIntegerOverflow=off
  Divide : Product  Inputs=*/
  Gain : Gain  Gain=100
  Product : Product
  Fx% : Outport
  wires:
  Gain/1 -> Abs/1
  <rMuX>/1 -> Product/1
  <Fz>/1 -> Add Constant/1
  <Fx>/1 -> Divide/1
  Product/1 -> Divide/2
  Divide/1 -> Gain/1
  Abs/1 -> Fx%/1
  Add Constant/1 -> Product/2

== system sm_car_/Scopes/Longitudinal Tire Usage/RR_X ==
  <Fx> : Inport
  <rMuX> : Inport  Port=2
  <Fz> : Inport  Port=3
  Abs : Abs  SaturateOnIntegerOverflow=off
  Add Constant : Bias  Bias=0.01  SaturateOnIntegerOverflow=off
  Divide : Product  Inputs=*/
  Gain : Gain  Gain=100
  Product : Product
  Fx% : Outport
  wires:
  Add Constant/1 -> Product/2
  Abs/1 -> Fx%/1
  Divide/1 -> Gain/1
  Product/1 -> Divide/2
  <Fx>/1 -> Divide/1
  <Fz>/1 -> Add Constant/1
  <rMuX>/1 -> Product/1
  Gain/1 -> Abs/1

== system sm_car_/Scopes/Stability Factor/Understeer Gradient Calculation ==
  VehBus : Inport
  Enable : EnablePort
  Add1 : Sum  Inputs=-+
  Bus Selector1 : BusSelector  OutputSignals=Chassis.SuspA1.Steer.aWheel,Chassis.Body.CG.vx,Chassis.Body.CG.nYaw,Chassis.Body.CG.gy
  Divide4 : Product  Inputs=/*
  Gain : Gain  Gain=1.575
  Gain1 : Gain  Gain=1/5.71
  Gain6 : Gain  Gain=1/9.81
  Product8 : Product  Inputs=*/
  K : Outport
  wires:
  VehBus/1 -> Bus Selector1/1
  Bus Selector1/1 -> Gain1/1  "<aWheel>"
  Bus Selector1/3 -> Divide4/2  "<nYaw>"
  Divide4/1 -> Gain/1
  Product8/1 -> K/1  "K"
  Gain/1 -> Add1/2
  Bus Selector1/2 -> Divide4/1  "<vx>"
  Bus Selector1/4 -> Gain6/1  "<gy>"
  Gain1/1 -> Add1/1
  Gain6/1 -> Product8/2
  Add1/1 -> Product8/1

== system sm_car_/Scopes/Yaw Reference/Subsystem ==
  v_x : Inport
  aSteerWheel : Inport  Port=2
  a_y : Inport  Port=3
  Enable : EnablePort
  Abs : Abs  SaturateOnIntegerOverflow=off
  Add : Sum
  Add Constant : Bias  Bias=1e-3  SaturateOnIntegerOverflow=off
  Divide : Product  Inputs=/*
  Divide1 : Product  Inputs=**/
  Gain : Gain  Gain=-0.00012434
  Gain1 : Gain  Gain=-1
  Power : Math  Operator=square
  Saturation Dynamic : sl_discontinuities/Saturation Dynamic  OutMin=[]  OutMax=[]  OutDataTypeStr=Inherit: Same as second input  OutDataType=fixdt(1, 16)  OutScaling=2^-10  DoSatur=off
  StrWheelRatio : Gain  Gain=1/5.71
  Wheelbase : Constant  Value=1.578
  y : Outport
  wires:
  Saturation Dynamic/1 -> y/1
  aSteerWheel/1 -> StrWheelRatio/1
  StrWheelRatio/1 -> Divide1/1  "aWheel_rad"
  Divide1/1 -> Saturation Dynamic/2  "YawDesired"
  v_x/1 -> Power/1, Divide1/2, Add Constant/1
  Power/1 -> Gain/1
  Gain1/1 -> Saturation Dynamic/3
  Gain/1 -> Add/1
  Divide/1 -> Abs/1
  Wheelbase/1 -> Add/2
  Add/1 -> Divide1/3
  Abs/1 -> Gain1/1, Saturation Dynamic/1  "YawMax"
  a_y/1 -> Divide/2
  Add Constant/1 -> Divide/1
